simulink model "Lab4_Task_1_final"  (R2025b)
settings: Solver=FixedStepAuto  StartTime=0.0  StopTime=inf  RelTol=1e-3
model workspace (MAT data in the model file):
  SL_ROS_VariableLengthArrays_MaxSizes.CommonInfo.ArrayTruncateAction = 'EmitWarning'
  SL_ROS_VariableLengthArrays_MaxSizes.MsgTypeMap = containers.Map
  SL_ROS_VariableLengthArrays_MaxSizes.MsgTypeMap.serialization.keys = {'sensor_msgs/LaserScan'}
  SL_ROS_VariableLengthArrays_MaxSizes.MsgTypeMap.serialization.values{1}(1).PropertyName = 'intensities'
  SL_ROS_VariableLengthArrays_MaxSizes.MsgTypeMap.serialization.values{1}(1).DataType = 'single'
  SL_ROS_VariableLengthArrays_MaxSizes.MsgTypeMap.serialization.values{1}(1).MaxLength = 360
  SL_ROS_VariableLengthArrays_MaxSizes.MsgTypeMap.serialization.values{1}(2).PropertyName = 'ranges'
  SL_ROS_VariableLengthArrays_MaxSizes.MsgTypeMap.serialization.values{1}(2).DataType = 'single'
  SL_ROS_VariableLengthArrays_MaxSizes.MsgTypeMap.serialization.values{1}(2).MaxLength = 360
  SL_ROS_VariableLengthArrays_MaxSizes.MsgTypeMap.serialization.uniformity = 0
  SL_ROS_VariableLengthArrays_MaxSizes.MsgTypeMap.serialization.keyType = 'char'
  SL_ROS_VariableLengthArrays_MaxSizes.MsgTypeMap.serialization.valueType = 'any'
undefined symbols (not defined in the file or in its folder): header, twist
libraries: ros2lib x4
settings Model: Creator=scott  LastModifiedBy=abodynasser22
settings OptimizationCC: DefaultParameterBehavior=Inlined  EnhancedBackFolding=on  PassReuseOutputArgsAs=Individual arguments  ZeroExternalMemoryAtStartup=off  ZeroInternalMemoryAtStartup=off  MaxStackSize=64  OptimizeBlockOrder=speed  DifferentSizesBufferReuse=on  OptimizationCustomize=off  EfficientTunableParamExpr=on
settings DebuggingCC: ParameterTunabilityLossMsg=error
settings HardwareCC: ProdBitPerPointer=32.0  ProdBitPerSizeT=32.0  ProdBitPerPtrDiffT=32.0  ProdWordSize=32.0  ProdHWDeviceType=Intel->x86-32 (Windows32)  UseEmbeddedCoderFeatures=off
settings SFSimCC: MATLABDynamicMemAlloc=off
settings RTWCC: SystemTargetFile=ert.tlc  HardwareBoard=Robot Operating System 2 (ROS 2)  TLCOptions="-aInlineSetEventsForThisBaseRateFcn=TLC_FALSE -aSuppressMultiTaskScheduler=TLC_FALSE  -aRateBasedStepFcn=0"  TemplateMakefile=ert_default_tmf  Toolchain=Colcon Tools  TargetLang=C++  Description=Embedded Coder
settings CodeAppCC: ForceParamTrailComments=on  IgnoreCustomStorageClasses=off  OperatorAnnotations=on  SimulinkDataObjDesc=on  SFDataObjDesc=on  InsertBlockDesc=on
settings ERTTargetCC: ExtModeTransport=2.0  ExtModeStaticAlloc=on  ExtModeAutomaticAllocSize=off  ExtModeMexFile=ext_xcp  ExtModeIntrfLevel=Level2 - Open  RootIOFormat=Structure reference  CodeInterfacePackaging=C++ class  SupportNonInlinedSFcns=on

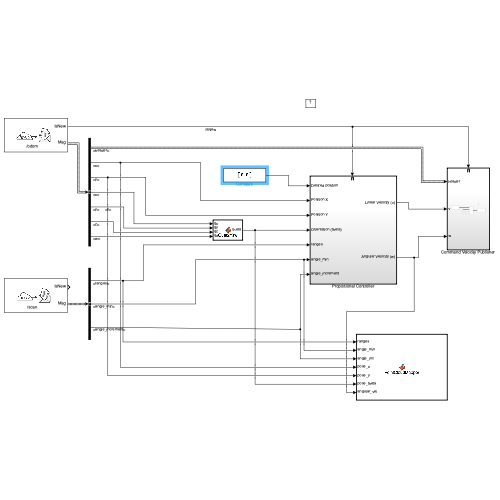
[thumbnail: Simulink's stored preview of the top-level diagram]
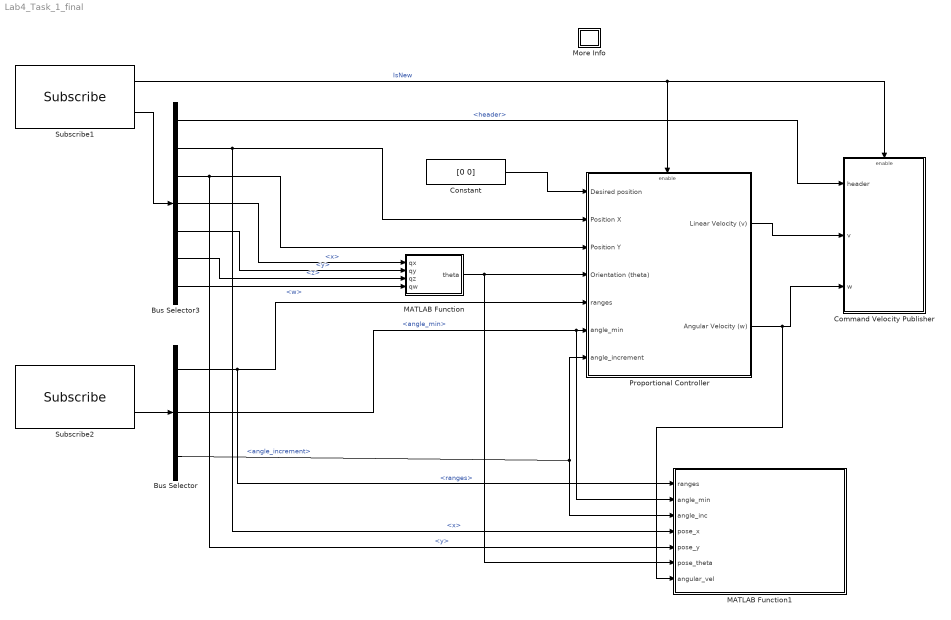
== system Lab4_Task_1_final ==
  Bus Selector : BusSelector  OutputSignals=ranges,angle_min,angle_increment
  Bus Selector3 : BusSelector  OutputSignals=header,pose.pose.position.x,pose.pose.position.y,pose.pose.orientation.x,pose.pose.orientation.y,pose.pose.orientation.z,pose.pose.orientation.w
  Command Velocity Publisher : Subsystem
  Constant : Constant  Value=[0 0]
  MATLAB Function : MATLAB Function  TreatAsAtomicUnit=on
  MATLAB Function1 : MATLAB Function  TreatAsAtomicUnit=on
  More Info : Subsystem
      settings: OpenFcn=showdemo(bdroot(gcb))
      mask Display: disp('?')
  Proportional Controller : Subsystem
  Subscribe1 : ros2lib/Subscribe  topicSource=Select from ROS network  topic=/odom  messageType=nav_msgs/Odometry  sampleTime=-1  QOSHistory=Keep last  QOSDepth=10  QOSReliability=Reliable  QOSDurability=Volatile  QOSDeadline=Inf  QOSLifespan=Inf  QOSLiveliness=Automatic  QOSLeaseDuration=Inf  QOSAvoidROSNamespaceConventions=off
  Subscribe2 : ros2lib/Subscribe  topicSource=Select from ROS network  topic=/scan  messageType=sensor_msgs/LaserScan  sampleTime=-1  QOSHistory=Keep last  QOSDepth=10  QOSReliability=Best effort  QOSDurability=Volatile  QOSDeadline=Inf  QOSLifespan=Inf  QOSLiveliness=Automatic  QOSLeaseDuration=Inf  QOSAvoidROSNamespaceConventions=off
  wires:
  Subscribe1/2 -> Bus Selector3/1
  Subscribe1/1 -> Command Velocity Publisher/Enable, Proportional Controller/Enable  "IsNew"
  Proportional Controller/1(Linear Velocity (v)) -> Command Velocity Publisher/2(v)
  Proportional Controller/2(Angular Velocity (w)) -> MATLAB Function1/7(angular_vel), Command Velocity Publisher/3(w)
  Bus Selector3/1 -> Command Velocity Publisher/1(header)  "<header>"
  Bus Selector3/2 -> MATLAB Function1/4(pose_x), Proportional Controller/2(Position X)  "<x>"
  Bus Selector3/3 -> MATLAB Function1/5(pose_y), Proportional Controller/3(Position Y)  "<y>"
  Bus Selector3/5 -> MATLAB Function/2(qy)  "<y>"
  Bus Selector3/6 -> MATLAB Function/3(qz)  "<z>"
  Subscribe2/2 -> Bus Selector/1
  Bus Selector/1 -> MATLAB Function1/1(ranges), Proportional Controller/5(ranges)  "<ranges>"
  Bus Selector/2 -> MATLAB Function1/2(angle_min), Proportional Controller/6(angle_min)  "<angle_min>"
  Bus Selector/3 -> MATLAB Function1/3(angle_inc), Proportional Controller/7(angle_increment)  "<angle_increment>"
  Bus Selector3/7 -> MATLAB Function/4(qw)  "<w>"
  MATLAB Function/1(theta) -> MATLAB Function1/6(pose_theta), Proportional Controller/4(Orientation (theta))
  Bus Selector3/4 -> MATLAB Function/1(qx)  "<x>"
  Constant/1 -> Proportional Controller/1(Desired position)

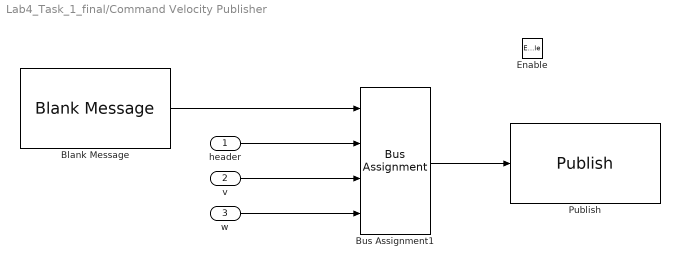
== system Lab4_Task_1_final/Command Velocity Publisher ==
  header : Inport
  v : Inport  Port=2
  w : Inport  Port=3
  Enable : EnablePort
  Blank Message : ros2lib/Blank Message  messageClass=Message  entityType=geometry_msgs/TwistStamped  messageType=geometry_msgs/TwistStamped  SampleTime=inf
  Bus Assignment1 : BusAssignment  DialogController=Simulink.DDGSource_BusAssignment  AssignedSignals=header,twist.linear.x,twist.angular.z
  Publish : ros2lib/Publish  topicSource=Select from ROS network  topic=/cmd_vel  messageType=geometry_msgs/TwistStamped  QOSHistory=Keep last  QOSDepth=10  QOSReliability=Reliable  QOSDurability=Volatile  QOSDeadline=Inf  QOSLifespan=Inf  QOSLiveliness=Automatic  QOSLeaseDuration=Inf  QOSAvoidROSNamespaceConventions=off
  wires:
  Bus Assignment1/1 -> Publish/1
  Blank Message/1 -> Bus Assignment1/1
  header/1 -> Bus Assignment1/2
  v/1 -> Bus Assignment1/3
  w/1 -> Bus Assignment1/4

== system Lab4_Task_1_final/More Info ==

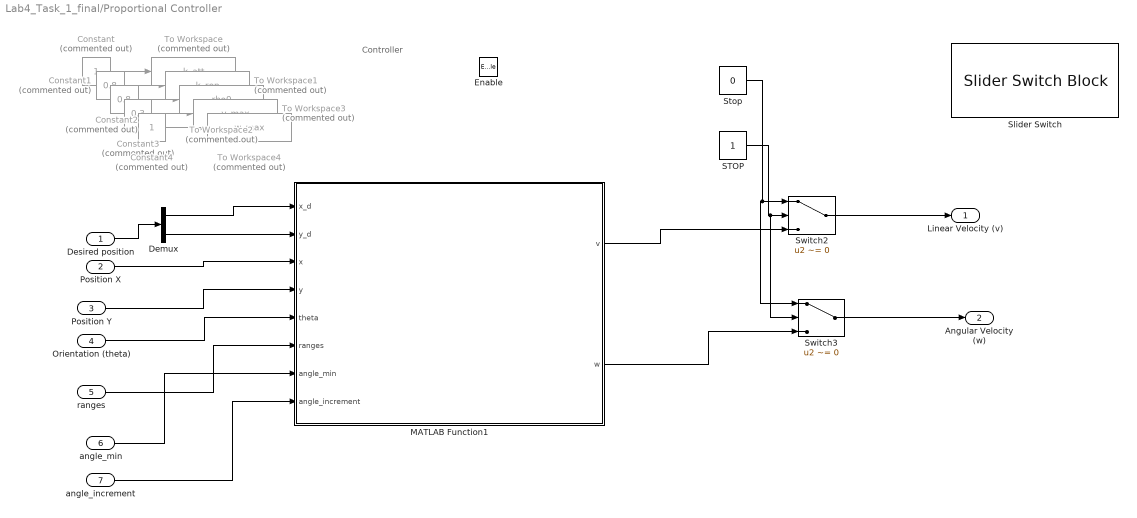
== system Lab4_Task_1_final/Proportional Controller ==
  note: Controller
  Desired position : Inport
  Position X : Inport  Port=2
  Position Y : Inport  Port=3
  Orientation (theta) : Inport  Port=4
  ranges : Inport  Port=5
  angle_min : Inport  Port=6
  angle_increment : Inport  Port=7
  Enable : EnablePort
  Constant : Constant  Commented=on
  Constant1 : Constant  Commented=on  Value=0.8
  Constant2 : Constant  Commented=on  Value=0.8
  Constant3 : Constant  Commented=on  Value=0.3
  Constant4 : Constant  Commented=on
  Demux : Demux  Outputs=2
  MATLAB Function1 : MATLAB Function  TreatAsAtomicUnit=on
  "STOP " : Constant
  Slider Switch : SliderSwitchBlock
  Stop : Constant  Value=0
  Switch2 : Switch  Criteria=u2 ~= 0  SaturateOnIntegerOverflow=off  InputSameDT=off
  Switch3 : Switch  Criteria=u2 ~= 0  SaturateOnIntegerOverflow=off  InputSameDT=off
  To Workspace : ToWorkspace  Commented=on  VariableName=k_att  SaveFormat=Timeseries  SampleTime=-1
  To Workspace1 : ToWorkspace  Commented=on  VariableName=k_rep  SaveFormat=Timeseries  SampleTime=-1
  To Workspace2 : ToWorkspace  Commented=on  VariableName=rho0  SaveFormat=Timeseries  SampleTime=-1
  To Workspace3 : ToWorkspace  Commented=on  VariableName=v_max  SaveFormat=Timeseries  SampleTime=-1
  To Workspace4 : ToWorkspace  Commented=on  VariableName=w_max  SaveFormat=Timeseries  SampleTime=-1
  Linear Velocity (v) : Outport  VectorParamsAs1DForOutWhenUnconnected=off
  Angular Velocity (w) : Outport  Port=2  VectorParamsAs1DForOutWhenUnconnected=off
  wires:
  Stop/1 -> Switch3/1, Switch2/1
  "STOP "/1 -> Switch3/2, Switch2/2
  Switch2/1 -> Linear Velocity (v)/1
  Switch3/1 -> Angular Velocity (w)/1
  MATLAB Function1/1(v) -> Switch2/3
  MATLAB Function1/2(w) -> Switch3/3
  Constant/1 -> To Workspace/1
  Constant1/1 -> To Workspace1/1
  Constant2/1 -> To Workspace2/1
  Constant3/1 -> To Workspace3/1
  Constant4/1 -> To Workspace4/1
  Desired position/1 -> Demux/1
  Demux/1 -> MATLAB Function1/1(x_d)
  Demux/2 -> MATLAB Function1/2(y_d)
  Position X/1 -> MATLAB Function1/3(x)
  Position Y/1 -> MATLAB Function1/4(y)
  Orientation (theta)/1 -> MATLAB Function1/5(theta)
  ranges/1 -> MATLAB Function1/6(ranges)
  angle_min/1 -> MATLAB Function1/7(angle_min)
  angle_increment/1 -> MATLAB Function1/8(angle_increment)

== matlab function Lab4_Task_1_final/MATLAB Function ==
  data: qx input; theta output; qy input; qz input; qw input
function theta = Quat2Yaw(qx, qy, qz, qw)
%#codegen
% Inputs are quaternion components from /odom:
% orientation.x = qx, .y = qy, .z = qz, .w = qw

% Build 1x4 quaternion row in the order [w x y z]
q = [qw, qx, qy, qz];

% Convert to Euler angles [yaw pitch roll] (ZYX convention)
eul = quat2eul(q, 'ZYX');

% Use yaw (rotation about Z-axis)
theta = eul(1);
end

== matlab function Lab4_Task_1_final/MATLAB Function1 ==
  data: ranges input; angle_min input; angle_inc input; pose_x input; pose_y input; pose_theta input; angular_vel input
function PointCloudMapper(ranges, angle_min, angle_inc, pose_x, pose_y, pose_theta, angular_vel)
    %#codegen
    
    % Persistent storage för point cloud och robot trail
    persistent cloud_x cloud_y
    persistent trail_x trail_y
    persistent update_count
    persistent last_plot_time
    
    % Initialisering
    if isempty(cloud_x)
        cloud_x = zeros(100000, 1);
        cloud_y = zeros(100000, 1);
        trail_x = zeros(5000, 1);
        trail_y = zeros(5000, 1);
        update_count = uint32(0);
        last_plot_time = 0;
    end
    
    % Skippa om roboten snurrar för snabbt (förhindrar ghost points)
    if abs(angular_vel) > 0.6
        return;
    end
    
    update_count = update_count + 1;
    
    % --- LIDAR TRANSFORMATION ---
    ranges = double(ranges(:));
    N = length(ranges);
    
    % Beräkna vinklar
    angles = double(angle_min) + (0:N-1)' * double(angle_inc);
    
    % Filtrera giltiga punkter
    valid = isfinite(ranges) & (ranges > 0.12) & (ranges < 3.5);
    
    if sum(valid) < 5
        return; % För få punkter
    end
    
    valid_ranges = ranges(valid);
    valid_angles = angles(valid);
    
    % Konvertera till robot frame (polar -> cartesian)
    robot_x = valid_ranges .* cos(valid_angles);
    robot_y = valid_ranges .* sin(valid_angles);
    
    % Transformera till world frame
    cos_theta = cos(pose_theta);
    sin_theta = sin(pose_theta);
    
    world_x = pose_x + robot_x * cos_theta - robot_y * sin_theta;
    world_y = pose_y + robot_x * sin_theta + robot_y * cos_theta;
    
    % Lägg till punkter i cloud (circular buffer)
    n_new = length(world_x);
    start_idx = mod(double(update_count) * 200, 100000) + 1;
    end_idx = min(start_idx + n_new - 1, 100000);
    actual_n = end_idx - start_idx + 1;
    
    cloud_x(start_idx:end_idx) = world_x(1:actual_n);
    cloud_y(start_idx:end_idx) = world_y(1:actual_n);
    
    % Lägg till robot position i trail
    trail_idx = mod(double(update_count), 5000) + 1;
    trail_x(trail_idx) = pose_x;
    trail_y(trail_idx) = pose_y;
    
    % --- PLOTTING ---
    % Plotta var 15:e uppdatering för bättre performance
    current_time = double(update_count);
    if (current_time - last_plot_time) >= 15
        last_plot_time = current_time;
        
        % Skapa/uppdatera figure
        fig = figure(99);
        clf(fig);
        hold on;
        
        % Plotta LIDAR points (blå, små, transparent)
        valid_cloud = (cloud_x ~= 0) | (cloud_y ~= 0);
        if sum(valid_cloud) > 0
            scatter(cloud_x(valid_cloud), cloud_y(valid_cloud), 1, 'b.', ...
                'MarkerEdgeAlpha', 0.3);
        end
        
        % Plotta robot trajectory (röd linje)
        valid_trail = (trail_x ~= 0) | (trail_y ~= 0);
        if sum(valid_trail) > 1
            plot(trail_x(valid_trail), trail_y(valid_trail), 'r-', 'LineWidth', 2);
        end
        
        % Markera start (gul) och slut (blå)
        trail_indices = find(valid_trail);
        if ~isempty(trail_indices)
            start_idx_trail = trail_indices(1);
            end_idx_trail = trail_indices(end);
            
            plot(trail_x(start_idx_trail), trail_y(start_idx_trail), 'yo', ...
                'MarkerSize', 8, 'MarkerFaceColor', 'y');
            plot(trail_x(end_idx_trail), trail_y(end_idx_trail), 'bo', ...
                'MarkerSize', 8, 'MarkerFaceColor', 'b');
        end
        
        % Formatering
        axis equal;
        grid on;
        xlabel('X (cm)');
        ylabel('Y (cm)');
        title('Following a wall');
        
        % Legend
        legend({'', 'Robots trajectory', 'Start', 'End'}, 'Location', 'best');
        
        % Invertera Y-axeln för att matcha din väns plot
        set(gca, 'YDir', 'reverse');
        
        drawnow limitrate;
    end
end

== matlab function Lab4_Task_1_final/Proportional Controller/MATLAB Function1 ==
  data: x_d input; y_d input; v output; x input; y input; theta input; ranges input; angle_min input; angle_increment input; w output
function [v, w] = PotentialFieldController(x_d, y_d, x, y, theta, ...
                                           ranges, angle_min, angle_increment)
%#codegen
% Tuned for Narrow Maze (0.4m corridors)
% Version: 2.0 (Tight Squeeze Edition)

% --- TUNED CONSTANTS ---
% Increased attraction to pull through narrow gaps
k_att = 1.8;      

% Decreased repulsion gain to prevent bouncing in tight spaces
k_rep = 0.4;      

% CRITICAL: Reduced range. 
% Must be < 0.2m (half of 0.4m corridor) to allow passage center.
rho0  = 0.25;      

% Slower speed for precision maneuvering
v_const = 0.12;    

% Max rotation speed
w_max = 0.4;      

% --- DEBUGGING ---
persistent tick
if isempty(tick), tick = 0; end
tick = tick + 1;
do_print = (mod(tick, 20) == 0);

% --- 0. DATA SANITIZATION ---
x_d = double(x_d); y_d = double(y_d);
x = double(x); y = double(y); theta = double(theta);
angle_min = double(angle_min); angle_increment = double(angle_increment);
ranges = double(ranges(:)); 
N = numel(ranges);

% --- 1. ATTRACTION FORCE ---
ex = x_d - x;
ey = y_d - y;
dist_goal = sqrt(ex^2 + ey^2);

% Loosened goal threshold slightly to prevent "hunting" at end
if dist_goal < 0.15
    v = 0.0; w = 0.0;
    if do_print, fprintf('GOAL REACHED! Dist: %.3f\n', dist_goal); end
    return;
end

F_att_x = k_att * (ex / dist_goal);
F_att_y = k_att * (ey / dist_goal);

% --- 2. REPULSION FORCE ---
F_rep_x = 0.0;
F_rep_y = 0.0;

angles_local = angle_min + (0:N-1)' * angle_increment;

% Filter valid ranges
valid_idx = (ranges > 0.05) & (ranges < rho0) & ~isinf(ranges);

if any(valid_idx)
    r_vals = ranges(valid_idx);        
    a_vals = angles_local(valid_idx);  
    
    alpha = theta + a_vals;
    
    % Magnitude
    % Note: 1/r^2 grows huge very fast. Lower k_rep balances this.
    raw_coeff = k_rep * (1./r_vals - 1/rho0) .* (1./r_vals.^2);
    
    % Cap extreme forces to prevent Simulink instability
    coeff = min(raw_coeff, 10.0);
    
    % Vectors
    c_alpha = cos(alpha);
    s_alpha = sin(alpha);
    
    dir_rep_x = -c_alpha;
    dir_rep_y = -s_alpha;
    
    % Tangential Swirl (Helps slide along walls)
    dir_tan_x = -s_alpha;
    dir_tan_y = c_alpha;
    
    % Mix: 30% Push, 70% Slide (Better for corridors)
    final_dir_x = 0.3 * dir_rep_x + 0.7 * dir_tan_x;
    final_dir_y = 0.3 * dir_rep_y + 0.7 * dir_tan_y;
    
    F_rep_x = sum(coeff .* final_dir_x);
    F_rep_y = sum(coeff .* final_dir_y);
end

% --- 3. TOTAL FORCE ---
Fx = F_att_x + F_rep_x;
Fy = F_att_y + F_rep_y;

% --- 4. KINEMATICS ---
psi_des = atan2(Fy, Fx);
e_psi = atan2(sin(psi_des - theta), cos(psi_des - theta));

% --- 5. VELOCITY LOGIC ---
current_v = v_const;
current_w_gain = 1.2; % Increased gain for sharper turns

% Slow down if repulsion is high (we are in a tight spot)
repulsion_mag = sqrt(F_rep_x^2 + F_rep_y^2);
if repulsion_mag > 1.0
    current_v = v_const * 0.5; % Crawl speed
end

% Slow down for heading errors
if abs(e_psi) > 0.5
    current_v = min(current_v, v_const * 0.3);
end

% STAGNATION RECOVERY
% If forces cancel out perfectly (Deadlock), nudge forward
if (abs(Fx) < 0.1 && abs(Fy) < 0.1)
    current_v = v_const * 0.8; % Force forward movement
    if do_print, fprintf('DEADLOCK DETECTED - FORCING MOVE\n'); end
end

% --- CONTROLLERS ---
v = current_v;
w = current_w_gain * e_psi;

% Saturation
if w > w_max, w = w_max; elseif w < -w_max, w = -w_max; end

% --- DEBUG ---
if do_print
    fprintf('D:%.2f | Att:[%.1f] | Rep:[%.1f] | Err:%.2f | v:%.2f\n', ...
        dist_goal, sqrt(F_att_x^2+F_att_y^2), repulsion_mag, e_psi, v);
end
end
